simulink model "ASM_Traffic_MultiCore"  (R2026a)
settings: Solver=ode1  StartTime=SIM.tstart.v  StopTime=SIM.tend.v  FixedStep=SIM.StepSize.v
PostLoadFcn:
  | if any(exist('dsrtsu_mdlpostloadfcn', 'file') ~= 0), dsrtsu_mdlpostloadfcn('Execute', bdroot); end
  | try, asm_mdl_postloadfcn(bdroot, 'UpdateModel', 3600); catch, disp(lasterr); end,
InitFcn:
  | , if any(exist('rtifpga_mdlclblib', 'file') ~= 0), rtifpga_mdlclblib('Init', bdroot); end,
  | , if any(exist('dsmpb_private', 'file') ~= 0), dsmpb_private('dsmpb_mdlclblib', 'Init', bdroot); end,
model workspace (MAT data in the model file):
  asmReferencePath = [0 0.01 0.02 0.03 0.04 0.05 0.06 0.07 0.08 0.09 0.1 0.11 ... (350007 elements, 50001x7)]
  roadBounds : Simulink.Parameter (value not decoded)
  safetyAxes : Simulink.Parameter (value not decoded)
undefined symbols (not defined in the file): _to_, a0b2, ASM_BrakeHydraulics_DemoSystems, ASM_VehicleDynamics_DemoSystems, b98103fe8ad365046cd0, BrakeCircuit, controllerConfig, CPT, Crankshaft, DiscIntNeverNeededParam, dsmsi, FinalDriveAssembly, MDL, ModeSignals, mu, Pos_BrakePedal_Maneuver, rad, RefSignals, roadFamilyData, roadFamilyId, s_to_rpm, SIM, SoftECU, Suspension, Tire, Transmission
libraries: ASM_Traffic_lib x135, simulink x98, ASM_Utils_lib x77, ASM_VehicleDynamics_lib x70, ASM_Environment_lib x22, dsmpblib x20, dsmsilib x15, MDLD_Utils_lib x10, ASM_BrakeHydraulics_lib x3, sl_discontinuities x2
(part 2 of 65)

== system ASM_Traffic_MultiCore/ASMTools ==
  note: ---- Code Generation ----
  note: ------ Multi-Instance ------
  note: ----- Scope Handling ------
  note: ----- Signal Handling ------
  note: ------------------- Project & Experiment Handling -------------------
  note: -------------------- ModelDesk Parameter Group --------------------
  note: ------------------------------- Tire Handling -------------------------------
  ASMSignalInterface_Manager : MDLD_Utils_lib/ModelDeskPlotInterface/ASMSignalInterface_Manager
  ASM_Model_Port_Manager : ASM_Utils_lib/Miscellaneous/ASM_MODEL_PORT_MANAGER
  GenerateVEOS : ASM_Utils_lib/CodeGeneration/GenerateVEOS
  ModelDeskParaGroupOverview : ASM_Utils_lib/ModelDeskInterface/ModelDeskParaGroupOverview
  MultiInstanceOverview : ASM_Utils_lib/ModelDeskInterface/MultiInstanceOverview
  OpenExperimentModelDesk : ASM_Utils_lib/OpenExperiment/OpenExperiment  ExpDir=..\Parameterization\MOD_Traffic\Experiment_001\Experiment_001.CDE  dSProduct=ModelDesk
  ReplaceTire : ASM_Utils_lib/BlockReplacement/ReplaceVariants  editSearchPath=bdroot  popupLibBlk=<select here>  popupTargetDemo=<select here>  Demosystem=VehicleDynamics_Tire  variantLib=ASM_VehicleDynamics_DemoSystems/Tire
  ScopeHandlingGui : ASM_Utils_lib/ReplaceScopes/ScopeHandlingGui

== system ASM_Traffic_MultiCore/AnimationInterface ==
  note: Animation Interface
  In : Inport
  ANIMATION_INTERFACE : Subsystem
  Bus Selector : BusSelector  OutputSignals=Environment.Animation.Sw_AnimationInterface[0Disabled|1Enabled],Environment.Animation.ManeuverState[]
  DriverAssistance_Animation : BusSelector  OutputSignals=DomainControl.DriverAssistance.Animation  OutputAsBus=on
  Drivetrain_Animation : BusSelector  OutputSignals=Drivetrain.Animation  OutputAsBus=on
  Environment_Animation : BusSelector  OutputSignals=Environment.Animation  OutputAsBus=on
  FcnCall : Subsystem
  Fellow_Doors : Subsystem
  Fellow_Lights : Subsystem
  OpenAnimationInterfaceModel : Subsystem
      settings: OpenFcn=|
      | InterfaceModel = 'ASM_AnimationInterface';
      | 
      | try
      |     open_system(InterfaceModel);                         catch
      |     errordlg(['ERROR opening Animation interface: ',InterfaceModel,'.slx']);
      | end
      mask Display: disp('Open ASM_AnimationInterface')
  Rate Transition{,1..3} (4 alike) : RateTransition  Integrity=off  OutPortSampleTimeOpt=Inherit
  VehicleDynamics_Animation : BusSelector  OutputSignals=VehicleDynamics.Animation  OutputAsBus=on
  Vehicle_Doors : Subsystem
  Vehicle_Lights : Subsystem
  wires:
  Bus Selector/1 -> FcnCall/Enable  "<Sw_AnimationInterface[0Disabled|1Enabled]>"
  Fellow_Doors/1(Fellow_Doors) -> ANIMATION_INTERFACE/8(Fellow_Doors)
  Vehicle_Doors/1(ASM_Vehicle_Doors) -> ANIMATION_INTERFACE/7(ASM_Vehicle_Doors)
  Rate Transition2/1 -> ANIMATION_INTERFACE/4(Environment_Animation), Vehicle_Lights/2(Environment_Animation), Fellow_Doors/1(Environment_Animation), Vehicle_Doors/1(Environment_Animation), Fellow_Lights/1(Environment_Animation)
  Vehicle_Lights/1(ASM_Vehicle_Lights) -> ANIMATION_INTERFACE/5(ASM_Vehicle_Lights)
  Fellow_Lights/1(Fellow_Light) -> ANIMATION_INTERFACE/6(Fellow_Lights)
  Rate Transition3/1 -> ANIMATION_INTERFACE/3(VehicleDynamics_Animation), Vehicle_Lights/1(VehicleDynamics_Animation)
  FcnCall/1(FcnCallEvent[]) -> ANIMATION_INTERFACE/Trigger
  Bus Selector/2 -> FcnCall/1(ManeuverState[])  "<ManeuverState[]>"
  Drivetrain_Animation/1 -> Rate Transition1/1
  Rate Transition1/1 -> ANIMATION_INTERFACE/2(Drivetrain_Animation)
  Rate Transition/1 -> ANIMATION_INTERFACE/1(DriverAssistance_Animation)
  Environment_Animation/1 -> Rate Transition2/1
  DriverAssistance_Animation/1 -> Rate Transition/1
  VehicleDynamics_Animation/1 -> Rate Transition3/1
  In/1 -> VehicleDynamics_Animation/1, Environment_Animation/1, Drivetrain_Animation/1, DriverAssistance_Animation/1, Bus Selector/1

== system ASM_Traffic_MultiCore/DomainControl ==
  In : Inport
  Bus Creator : BusCreator  Inputs=3
  DriverAssistance : Subsystem
  StartSystem : Subsystem
  TorqueManager : Subsystem
  Out : Outport  VectorParamsAs1DForOutWhenUnconnected=off
  wires:
  Bus Creator/1 -> Out/1  "DomainControl"
  In/1 -> StartSystem/1(In), DriverAssistance/1(In), TorqueManager/1(In)
  DriverAssistance/1(Out) -> Bus Creator/3
  StartSystem/1(Out) -> Bus Creator/1
  TorqueManager/1(Out) -> Bus Creator/2

== system ASM_Traffic_MultiCore/Driver ==
  note: Driver
  In : Inport
  steering_wheel[deg] : Inport  Port=2
  Interface_In : Subsystem
  Interface_Out : Subsystem
  Plant : Subsystem
  SignalInterface : Subsystem
  Out : Outport  VectorParamsAs1DForOutWhenUnconnected=off
  wires:
  In/1 -> Interface_In/1(In)
  Interface_In/1(Out) -> SignalInterface/1(In), Plant/1(Interface_In)
  Plant/1(Plant) -> Interface_Out/1(In)
  Interface_Out/1(Out) -> Out/1
  steering_wheel[deg]/1 -> Plant/2(steering_wheel[deg])

== system ASM_Traffic_MultiCore/Drivetrain ==
  note: Drivetrain
  In : Inport
  drive_trq[Nm] : Inport  Port=2
  Bus Creator1 : BusCreator  Inputs=2
  Control : Subsystem
  Interface_In : Subsystem
  Interface_Out : Subsystem
  Plant : Subsystem
  SignalInterface : Subsystem
  Out : Outport  VectorParamsAs1DForOutWhenUnconnected=off
  wires:
  Control/1(Control) -> Plant/2(Control), Bus Creator1/2
  Plant/1(Plant) -> Control/2(Plant), Bus Creator1/1
  Bus Creator1/1 -> Interface_Out/1(In)
  In/1 -> Interface_In/1(In)
  Interface_Out/1(Out) -> Out/1
  Interface_In/1(Out) -> SignalInterface/1(In), Control/1(Interface_In), Plant/1(Interface_In)
  drive_trq[Nm]/1 -> Plant/3(drive_trq[Nm])

== system ASM_Traffic_MultiCore/ElectricalSystem ==
  note: Electrical System Basic
  In : Inport
  Bus Creator2 : BusCreator  Inputs=2
  Control : Subsystem
  Interface_In : Subsystem
  Interface_Out : Subsystem
  Plant : Subsystem
  SignalInterface : Subsystem
  Out : Outport  VectorParamsAs1DForOutWhenUnconnected=off
  wires:
  Bus Creator2/1 -> Interface_Out/1(In)
  Control/1(Control) -> Plant/2(Control), Bus Creator2/2
  In/1 -> Interface_In/1(In)
  Plant/1(Plant) -> Control/2(Plant), Bus Creator2/1
  Interface_Out/1(Out) -> Out/1
  Interface_In/1(Out) -> SignalInterface/1(In), Control/1(Interface_In), Plant/1(Interface_In)

== system ASM_Traffic_MultiCore/Engine ==
  note: Engine Basic
  In : Inport
  Bus Creator1 : BusCreator  Inputs=2
  Control : Subsystem
  Interface_In : Subsystem
  Interface_Out : Subsystem
  Plant : Subsystem
  SignalInterface : Subsystem
  Out : Outport  VectorParamsAs1DForOutWhenUnconnected=off
  wires:
  In/1 -> Interface_In/1(In)
  Interface_Out/1(Out) -> Out/1
  Control/1(Control) -> Plant/2(Control), Bus Creator1/2
  Interface_In/1(Out) -> SignalInterface/1(In), Control/1(Interface_In), Plant/1(Interface_In)
  Plant/1(Plant) -> Bus Creator1/1, Control/2(Plant)
  Bus Creator1/1 -> Interface_Out/1(In)

== system ASM_Traffic_MultiCore/Environment ==
  note: Environment Traffic
  In : Inport
  Bus Creator1 : BusCreator  Inputs=6
  GroundTruth : Subsystem
  Interface_In : Subsystem
  Interface_Out : Subsystem
  Maneuver : Subsystem
  ModelDesk_MC_ID_Environment : ASM_Utils_lib/ModelDeskInterface/ModelDesk_MC  Tag=ASM_MAINCOMPONENT  Editable=off  MainComponent=Environment
  Road : Subsystem
  Sensors : Subsystem
  SignalInterface : Subsystem
  Traffic : Subsystem
  Out : Outport  VectorParamsAs1DForOutWhenUnconnected=off
  wires:
  In/1 -> Interface_In/1(In)
  GroundTruth/1(Out) -> Bus Creator1/6
  Sensors/1(Out) -> Bus Creator1/5
  Interface_In/1(Out) -> Bus Creator1/1
  Bus Creator1/1 -> SignalInterface/1(In), Sensors/1(In), Traffic/1(In), Road/1(In), Maneuver/1(In), GroundTruth/1(In), Interface_Out/1(In)
  Traffic/1(Out) -> Bus Creator1/4
  Road/1(Out) -> Bus Creator1/3
  Maneuver/1(Out) -> Bus Creator1/2
  Interface_Out/1(Out) -> Out/1

== system ASM_Traffic_MultiCore/Help ==

== system ASM_Traffic_MultiCore/VehicleDynamics ==
  note: Vehicle Dynamics
  In : Inport
  Ext_BrakeTrq[Nm] : Inport  Port=2
  deltaF_cmd_deg : Inport  Port=3
  Bus Creator1 : BusCreator  Inputs=2
  Control : Subsystem
  Interface_In : Subsystem
  Interface_Out : Subsystem
  Plant : Subsystem
  SignalInterface : Subsystem
  Out : Outport  VectorParamsAs1DForOutWhenUnconnected=off
  F_y[N] : Outport  Port=2
  F_z[N] : Outport  Port=3
  wires:
  Interface_Out/1(Out) -> Out/1
  In/1 -> Interface_In/1(In)
  Plant/1(Plant) -> Bus Creator1/1, Control/2(Plant)
  Control/1(Control) -> Plant/4(Control), Bus Creator1/2
  Interface_In/1(Out) -> SignalInterface/1(In), Control/1(Interface_In), Plant/3(Interface_In)
  Bus Creator1/1 -> Interface_Out/1(In)
  Ext_BrakeTrq[Nm]/1 -> Plant/2(Ext_BrakeTrq[Nm])
  Plant/2(F_y[N]) -> F_y[N]/1
  Plant/3(F_z[N]) -> F_z[N]/1
  deltaF_cmd_deg/1 -> Plant/1(deltaF_cmd_deg)

== system ASM_Traffic_MultiCore/controller_subsys ==
  In Bus Element : Inport  PortName=measurements  Element=x
  BusElementIn2 : Inport  PortName=measurements  Element=vx
  BusElementIn : Inport  PortName=measurements  Element=s
  horizon_prep_in : Inport  Port=2
  fellow : Inport  Port=3
  In Bus Element2 : Inport  Port=4  PortName=execution
  Reshape : Reshape  OutputDimensionality=Customize  OutputDimensions=[205,1]
  Terminator : Terminator
  Unit Delay : UnitDelay  SampleTime=0.05
  Unit Delay1 : UnitDelay  SampleTime=0.05
  acados_solver : Subsystem
  assemble_problem : MATLAB Function  TreatAsAtomicUnit=on
  horizon_prep : MATLAB Function  TreatAsAtomicUnit=on
  input_prep : Subsystem
  output_routing : Subsystem
  warm_start : Subsystem
  Out Bus Element : Outport  PortName=command
  Out Bus Element1 : Outport  Port=2  PortName=telemetry
  wires:
  acados_solver/1(solver_outputs) -> output_routing/1(solver_outputs)
  In Bus Element/1 -> assemble_problem/1(x)
  assemble_problem/1(solverInputs) -> input_prep/1(InBus)
  output_routing/2(predictions) -> warm_start/1(predictions)
  warm_start/1(x_pred) -> Unit Delay/1
  warm_start/2(u_pred) -> Unit Delay1/1
  input_prep/1(solverInputs) -> acados_solver/1(solverInputs)  "replay"
  horizon_prep/1(P) -> assemble_problem/2(P)
  BusElementIn2/1 -> horizon_prep/2(vx)
  BusElementIn/1 -> horizon_prep/1(s)
  output_routing/1(command) -> Out Bus Element/1
  output_routing/3(telemetry) -> Out Bus Element1/1
  In Bus Element2/1 -> input_prep/2(InBus1)
  Unit Delay/1 -> assemble_problem/3(Xguess), Reshape/1
  Unit Delay1/1 -> assemble_problem/4(Uguess)
  Reshape/1 -> horizon_prep/4(Xguess)
  horizon_prep_in/1 -> Terminator/1
  fellow/1 -> horizon_prep/3(fellow)

== system ASM_Traffic_MultiCore/exec_setting ==
  Constant : Constant  Value=false  OutDataTypeStr=boolean
  Constant1 : Constant  Value=true  OutDataTypeStr=boolean
  Constant2 : Constant  Value=200
  Out Bus Element : Outport  PortName=execution  Element=reset
  BusElementOut : Outport  PortName=execution  Element=enable
  BusElementOut1 : Outport  PortName=execution  Element=cap
  wires:
  Constant/1 -> Out Bus Element/1
  Constant1/1 -> BusElementOut/1
  Constant2/1 -> BusElementOut1/1

== system ASM_Traffic_MultiCore/state_conversion ==
  In4 : Inport
  F_y[N] : Inport  Port=2
  F_z[N] : Inport  Port=3
  ASM_adapter : MATLAB Function  TreatAsAtomicUnit=on
  Angle_fl_fr_wheel_vector : Concatenate
  Bus Selector : BusSelector  OutputSignals=x,vx,s
  Constant : Constant  Value=0
  Gain : Gain  Gain=1/3.6
  Gain1 : Gain  Gain=1/3.6
  Horizon_prep_in_vector : Concatenate  NumInputs=4
  Kinematic_sI_vector : Concatenate  NumInputs=4
  Reference_SI_vector : Concatenate  NumInputs=7
  Terminator{,2,5..6} (4 alike) : Terminator
  deg2rad : Gain  Gain=pi/180
  deg2rad1 : Gain  Gain=pi/180
  deg2rad2 : Gain  Gain=pi/180
  fellow_vector : Concatenate  NumInputs=4
  measured_pos : Concatenate
  required_measurement : BusSelector  OutputSignals=VehicleDynamics.Plant.v_x_Vehicle_CoG[km|h],VehicleDynamics.Plant.v_y_Vehicle_CoG[km|h],VehicleDynamics.Plant.Angle_Yaw_Vehicle_CoorSys_E[deg],VehicleDynamics.Plant.YawRate_Vehicle_CoG[deg|s],VehicleDynamics.Plant.Pos_x_Vehicle_CoorSys_E[m],VehicleDynamics.Plant.Pos_y_Vehicle_CoorSys_E[m],VehicleDynamics.Plant.Angle_SteeringWheel[deg],Environment.Plant.Pos_x_Ref_Vehicle_Road[m],Environment.Plant.Pos_y_Ref_Vehicle_Road[m],Environment.Plant.Curv_Vehicle_Road[1|m],Environment.Plant.s_Total_Vehicle_Road[m],Environment.Plant.s_Vehicle_Road[m],Environment.Plant.Angle_Yaw_Veh_Road[deg],Environment.Plant.v_Vehicle_Ref_Maneuver[m|s],Environment.Plant.v_Vehicle_Preview_Ref_Maneuver[m|s],Environment.Plant.Curv_Preview_Road[1|m],Driver.Plant.s_Preview[m],Environment.Plant.Pos_y_Preview_Road[m],Environment.Plant.Pos_x_Preview_Road[m],Environment.Plant.d_Total_Fellows[m],Environment.Plant.s_Fellows_Ref[m],Environment.Animation.Flag_FellowUsed[0|1],Environment.Animation.v_Fellows[km|h],Environment.Plant.Fric_Coeff_CP[:][],VehicleDynamics.Plant.Trq_Max_Brake[Nm],VehicleDynamics.Animation.F_FL_Tire_CoorSys_V[x;y;z][N],VehicleDynamics.Animation.F_FR_Tire_CoorSys_V[x;y;z][N],VehicleDynamics.Animation.F_RL_Tire_CoorSys_V[x;y;z][N],VehicleDynamics.Animation.F_RR_Tire_CoorSys_V[x;y;z][N],VehicleDynamics.Animation.Angle_FL_Wheel[Toe;Camber][deg],VehicleDynamics.Animation.Angle_FR_Wheel[Toe;Camber][deg]
  tire_feature_vector : Concatenate  NumInputs=6
  BusElementOut : Outport  PortName=measurement  Element=x
  BusElementOut1 : Outport  PortName=measurement  Element=vx
  Out Bus Element : Outport  PortName=measurement  Element=s
  horizon_prep_in : Outport  Port=2
  fellow : Outport  Port=3
  FyWheel[N] : Outport  Port=4
  FzWheel : Outport  Port=5
  tire_feature : Outport  Port=6
  Angle_FL_FR_Wheel[Toe;Camber][deg] : Outport  Port=7
  wires:
  Gain1/1 -> Kinematic_sI_vector/2
  required_measurement/5 -> measured_pos/1  "<Pos_x_Vehicle_CoorSys_E[m]>"
  required_measurement/9 -> Reference_SI_vector/2  "<Pos_y_Ref_Vehicle_Road[m]>"
  required_measurement/7 -> Terminator/1  "<Angle_SteeringWheel[deg]>"
  deg2rad1/1 -> Kinematic_sI_vector/4
  required_measurement/3 -> deg2rad/1  "<Angle_Yaw_Vehicle_CoorSys_E[deg]>"
  measured_pos/1 -> ASM_adapter/2(vehicleXY)
  Gain/1 -> Kinematic_sI_vector/1
  Kinematic_sI_vector/1 -> ASM_adapter/1(kinematicsSI)
  required_measurement/4 -> deg2rad1/1  "<YawRate_Vehicle_CoG[deg|s]>"
  required_measurement/6 -> measured_pos/2  "<Pos_y_Vehicle_CoorSys_E[m]>"
  required_measurement/1 -> Gain/1  "<v_x_Vehicle_CoG[km|h]>"
  deg2rad/1 -> Kinematic_sI_vector/3
  ASM_adapter/1(measurement) -> Bus Selector/1
  required_measurement/2 -> Gain1/1  "<v_y_Vehicle_CoG[km|h]>"
  required_measurement/8 -> Reference_SI_vector/1  "<Pos_x_Ref_Vehicle_Road[m]>"
  In4/1 -> required_measurement/1
  Reference_SI_vector/1 -> ASM_adapter/3(referenceSI)
  Bus Selector/1 -> BusElementOut/1  "<x>"
  Bus Selector/2 -> BusElementOut1/1  "<vx>"
  Bus Selector/3 -> Out Bus Element/1  "<s>"
  required_measurement/12 -> Terminator2/1  "<s_Vehicle_Road[m]>"
  required_measurement/11 -> Reference_SI_vector/3  "<s_Total_Vehicle_Road[m]>"
  required_measurement/10 -> Reference_SI_vector/5  "<Curv_Vehicle_Road[1|m]>"
  required_measurement/19 -> Terminator6/1  "<Pos_x_Preview_Road[m]>"
  required_measurement/18 -> Terminator5/1  "<Pos_y_Preview_Road[m]>"
  required_measurement/16 -> Horizon_prep_in_vector/3  "<Curv_Preview_Road[1|m]>"
  required_measurement/13 -> deg2rad2/1  "<Angle_Yaw_Veh_Road[deg]>"
  required_measurement/14 -> Reference_SI_vector/7, Horizon_prep_in_vector/1  "<v_Vehicle_Ref_Maneuver[m|s]>"
  required_measurement/15 -> Horizon_prep_in_vector/2  "<v_Vehicle_Preview_Ref_Maneuver[m|s]>"
  Constant/1 -> Reference_SI_vector/6
  deg2rad2/1 -> Reference_SI_vector/4
  required_measurement/17 -> Horizon_prep_in_vector/4  "<s_Preview[m]>"
  Horizon_prep_in_vector/1 -> horizon_prep_in/1
  required_measurement/20 -> fellow_vector/1  "<d_Total_Fellows[m]>"
  required_measurement/21 -> fellow_vector/2  "<s_Fellows_Ref[m]>"
  required_measurement/22 -> fellow_vector/3  "<Flag_FellowUsed[0|1]>"
  required_measurement/23 -> fellow_vector/4  "<v_Fellows[km|h]>"
  fellow_vector/1 -> fellow/1
  required_measurement/24 -> tire_feature_vector/1  "<Fric_Coeff_CP[:][]>"
  required_measurement/25 -> tire_feature_vector/2  "<Trq_Max_Brake[Nm]>"
  required_measurement/26 -> tire_feature_vector/3  "<F_FL_Tire_CoorSys_V[x;y;z][N]>"
  required_measurement/27 -> tire_feature_vector/4  "<F_FR_Tire_CoorSys_V[x;y;z][N]>"
  required_measurement/28 -> tire_feature_vector/5  "<F_RL_Tire_CoorSys_V[x;y;z][N]>"
  required_measurement/29 -> tire_feature_vector/6  "<F_RR_Tire_CoorSys_V[x;y;z][N]>"
  tire_feature_vector/1 -> tire_feature/1
  F_z[N]/1 -> FzWheel/1
  F_y[N]/1 -> FyWheel[N]/1
  required_measurement/30 -> Angle_fl_fr_wheel_vector/1  "<Angle_FL_Wheel[Toe;Camber][deg]>"
  required_measurement/31 -> Angle_fl_fr_wheel_vector/2  "<Angle_FR_Wheel[Toe;Camber][deg]>"
  Angle_fl_fr_wheel_vector/1 -> Angle_FL_FR_Wheel[Toe;Camber][deg]/1

== system ASM_Traffic_MultiCore/telemetry_unwrapped ==
  In1 : Inport
  Bus Selector : BusSelector  OutputSignals=slack_values,solver_status,cost_value,kkt_residuals,cpu_time,cpu_time_qp,cpu_time_lin,sqp_iter,qp_iteration_history,residual_history,history_length,lam_stage0
  Terminator{,1..11} (12 alike) : Terminator
  history_length : SignalConversion  OverrideOpt=off
  kkt_residuals : SignalConversion  OverrideOpt=off
  lam_stage0 : SignalConversion  OverrideOpt=off
  linearization_time_s : SignalConversion  OverrideOpt=off
  qp_iteration_history : SignalConversion  OverrideOpt=off
  qp_time_s : SignalConversion  OverrideOpt=off
  residual_history : SignalConversion  OverrideOpt=off
  slack_values : SignalConversion  OverrideOpt=off
  solver_cost : SignalConversion  OverrideOpt=off
  solver_status : SignalConversion  OverrideOpt=off
  solver_time_s : SignalConversion  OverrideOpt=off
  sqp_iterations : SignalConversion  OverrideOpt=off
  wires:
  Bus Selector/1 -> slack_values/1  "<slack_values>"
  Bus Selector/9 -> qp_iteration_history/1  "<qp_iteration_history>"
  Bus Selector/12 -> lam_stage0/1  "<lam_stage0>"
  Bus Selector/10 -> residual_history/1  "<residual_history>"
  Bus Selector/11 -> history_length/1  "<history_length>"
  In1/1 -> Bus Selector/1
  Bus Selector/2 -> solver_status/1  "<solver_status>"
  solver_status/1 -> Terminator1/1  "solver_status"
  Bus Selector/3 -> solver_cost/1  "<cost_value>"
  solver_cost/1 -> Terminator2/1  "solver_cost"
  Bus Selector/4 -> kkt_residuals/1  "<kkt_residuals>"
  kkt_residuals/1 -> Terminator3/1  "kkt_residuals"
  Bus Selector/5 -> solver_time_s/1  "<cpu_time>"
  solver_time_s/1 -> Terminator4/1  "solver_time_s"
  Bus Selector/6 -> qp_time_s/1  "<cpu_time_qp>"
  qp_time_s/1 -> Terminator5/1  "qp_time_s"
  Bus Selector/7 -> linearization_time_s/1  "<cpu_time_lin>"
  linearization_time_s/1 -> Terminator6/1  "linearization_time_s"
  Bus Selector/8 -> sqp_iterations/1  "<sqp_iter>"
  sqp_iterations/1 -> Terminator7/1  "sqp_iterations"
  slack_values/1 -> Terminator/1  "slack_values"
  qp_iteration_history/1 -> Terminator8/1
  residual_history/1 -> Terminator9/1
  lam_stage0/1 -> Terminator11/1
  history_length/1 -> Terminator10/1

== system ASM_Traffic_MultiCore/AnimationInterface/ANIMATION_INTERFACE ==
  DriverAssistance_Animation : Inport
  Drivetrain_Animation : Inport  Port=2
  VehicleDynamics_Animation : Inport  Port=3
  Environment_Animation : Inport  Port=4
  ASM_Vehicle_Lights : Inport  Port=5
  Fellow_Lights : Inport  Port=6
  ASM_Vehicle_Doors : Inport  Port=7
  Fellow_Doors : Inport  Port=8
  function : TriggerPort  TriggerType=function-call  VariantControl=Variant
  ACC_Instruments : Subsystem  Tag=Animation_ACC_Instruments  Priority=10001  Commented=on
  ASM_Vehicle : Subsystem  Tag=Animation_ASM_Vehicle  Priority=10001
  ASM_Vehicle_Instruments : Subsystem  Tag=Animation_ASM_Vehicle_Instruments  Priority=10001
  ASM_Vehicle_Occupants : Subsystem  Tag=Animation_ASM_Vehicle_Occupants  Priority=10001
  Activate_Animation : Subsystem  mask{ASMVehicle=Uncomment, ASMVehicleInstruments=Uncomment, ASMSensors=Uncomment, BoundigBoxes=Uncomment}
      mask prompts: ASMVehicle "ASM Vehicle"; ASMVehicleInstruments "ASM Vehicle Instruments"; ASMSensors "ASM Sensors"; BoundigBoxes "Bounding Boxes"
      settings: OpenFcn=|
      | subsysTag = 'Animation_Bounding_Boxes';
      | subsys = find_system(get_param(gcb,'Parent'),'SearchDepth','1','IncludeCommented','on','Tag',subsysTag);
      | if ~isempty(subsys)
      |     subsysState = get_param(subsys,'commented');
      |     if strcmp(subsysState,'off')
      |         set_param(subsys{1},'commented','on')
      |     end
      |     if strcmp(subsysState,'on')
      |         set_param(subsys{1},'commented','off')
      |     end
      | else
      |     disp(['Subsystem tagged with ''', subsysTag, ''' could not be found. The button is without action.'])
      | end
      mask TypeOptions ASMVehicle: Comment out | Uncomment
      mask Callback ASMVehicle: asm_vehicle_comment(gcb)
      mask TypeOptions ASMVehicleInstruments: Comment out | Uncomment
      mask TypeOptions ASMSensors: Comment out | Uncomment
      mask Callback ASMSensors:
      | subsys = find_system(get_param(gcb,'Parent'),'SearchDepth','1','IncludeCommented','on','Tag','ASM_Sensors');
      | if ~isempty(subsys)
      |     button_state = get_param(gcb,'ASMSensors');
      |     subsys_state = get_param(subsys,'commented');
      |     if strcmp(button_state,'Comment out') && strcmp(subsys_state,'off')
      |         set_param(subsys{1},'commented','on')
      |     end
      |     if strcmp(button_state,'Uncomment') && strcmp(subsys_state,'on')
      |         set_param(subsys{1},'commented','off')
      |     end
      | end
      mask TypeOptions BoundigBoxes: Comment out | Uncomment
      mask Display: disp('double click to\n activate/deactivate')
  Activate_Animation1 : Subsystem  mask{ASMVehicle=Uncomment, ASMVehicleInstruments=Uncomment, ASMSensors=Uncomment, BoundigBoxes=Uncomment}
      mask prompts: ASMVehicle "ASM Vehicle"; ASMVehicleInstruments "ASM Vehicle Instruments"; ASMSensors "ASM Sensors"; BoundigBoxes "Bounding Boxes"
      settings: OpenFcn=|
      | subsysTag = 'Animation_Fellows';
      | subsys = find_system(get_param(gcb,'Parent'),'SearchDepth','1','IncludeCommented','on','Tag',subsysTag);
      | if ~isempty(subsys)
      |     subsysState = get_param(subsys,'commented');
      |     if strcmp(subsysState,'off')
      |         set_param(subsys{1},'commented','on')
      |     end
      |     if strcmp(subsysState,'on')
      |         set_param(subsys{1},'commented','off')
      |     end
      | else
      |     disp(['Subsystem tagged with ''', subsysTag, ''' could not be found. The button is without action.'])
      | end
      mask TypeOptions ASMVehicle: Comment out | Uncomment
      mask Callback ASMVehicle: asm_vehicle_comment(gcb)
      mask TypeOptions ASMVehicleInstruments: Comment out | Uncomment
      mask TypeOptions ASMSensors: Comment out | Uncomment
      mask Callback ASMSensors:
      | subsys = find_system(get_param(gcb,'Parent'),'SearchDepth','1','IncludeCommented','on','Tag','ASM_Sensors');
      | if ~isempty(subsys)
      |     button_state = get_param(gcb,'ASMSensors');
      |     subsys_state = get_param(subsys,'commented');
      |     if strcmp(button_state,'Comment out') && strcmp(subsys_state,'off')
      |         set_param(subsys{1},'commented','on')
      |     end
      |     if strcmp(button_state,'Uncomment') && strcmp(subsys_state,'on')
      |         set_param(subsys{1},'commented','off')
      |     end
      | end
      mask TypeOptions BoundigBoxes: Comment out | Uncomment
      mask Display: disp('double click to\n activate/deactivate')
  Activate_Animation2 : Subsystem  mask{ASMVehicle=Uncomment, ASMVehicleInstruments=Uncomment, ASMSensors=Uncomment, BoundigBoxes=Uncomment}
      mask prompts: ASMVehicle "ASM Vehicle"; ASMVehicleInstruments "ASM Vehicle Instruments"; ASMSensors "ASM Sensors"; BoundigBoxes "Bounding Boxes"
      settings: OpenFcn=|
      | subsysTag = 'Animation_Data_Streams_Instruments';
      | subsys = find_system(get_param(gcb,'Parent'),'SearchDepth','1','IncludeCommented','on','Tag',subsysTag);
      | if ~isempty(subsys)
      |     subsysState = get_param(subsys,'commented');
      |     if strcmp(subsysState,'off')
      |         set_param(subsys{1},'commented','on')
      |     end
      |     if strcmp(subsysState,'on')
      |         set_param(subsys{1},'commented','off')
      |     end
      | else
      |     disp(['Subsystem tagged with ''', subsysTag, ''' could not be found. The button is without action.'])
      | end
      mask TypeOptions ASMVehicle: Comment out | Uncomment
      mask Callback ASMVehicle: asm_vehicle_comment(gcb)
      mask TypeOptions ASMVehicleInstruments: Comment out | Uncomment
      mask TypeOptions ASMSensors: Comment out | Uncomment
      mask Callback ASMSensors:
      | subsys = find_system(get_param(gcb,'Parent'),'SearchDepth','1','IncludeCommented','on','Tag','ASM_Sensors');
      | if ~isempty(subsys)
      |     button_state = get_param(gcb,'ASMSensors');
      |     subsys_state = get_param(subsys,'commented');
      |     if strcmp(button_state,'Comment out') && strcmp(subsys_state,'off')
      |         set_param(subsys{1},'commented','on')
      |     end
      |     if strcmp(button_state,'Uncomment') && strcmp(subsys_state,'on')
      |         set_param(subsys{1},'commented','off')
      |     end
      | end
      mask TypeOptions BoundigBoxes: Comment out | Uncomment
      mask Display: disp('double click to\n activate/deactivate')
  Activate_Animation3 : Subsystem  mask{ASMVehicle=Uncomment, ASMVehicleInstruments=Uncomment, ASMSensors=Uncomment, BoundigBoxes=Uncomment}
      mask prompts: ASMVehicle "ASM Vehicle"; ASMVehicleInstruments "ASM Vehicle Instruments"; ASMSensors "ASM Sensors"; BoundigBoxes "Bounding Boxes"
      settings: OpenFcn=|
      | subsysTag = 'Animation_Lane_Sensor';
      | subsys = find_system(get_param(gcb,'Parent'),'SearchDepth','1','IncludeCommented','on','Tag',subsysTag);
      | if ~isempty(subsys)
      |     subsysState = get_param(subsys,'commented');
      |     if strcmp(subsysState,'off')
      |         set_param(subsys{1},'commented','on')
      |     end
      |     if strcmp(subsysState,'on')
      |         set_param(subsys{1},'commented','off')
      |     end
      | else
      |     disp(['Subsystem tagged with ''', subsysTag, ''' could not be found. The button is without action.'])
      | end
      mask TypeOptions ASMVehicle: Comment out | Uncomment
      mask Callback ASMVehicle: asm_vehicle_comment(gcb)
      mask TypeOptions ASMVehicleInstruments: Comment out | Uncomment
      mask TypeOptions ASMSensors: Comment out | Uncomment
      mask Callback ASMSensors:
      | subsys = find_system(get_param(gcb,'Parent'),'SearchDepth','1','IncludeCommented','on','Tag','ASM_Sensors');
      | if ~isempty(subsys)
      |     button_state = get_param(gcb,'ASMSensors');
      |     subsys_state = get_param(subsys,'commented');
      |     if strcmp(button_state,'Comment out') && strcmp(subsys_state,'off')
      |         set_param(subsys{1},'commented','on')
      |     end
      |     if strcmp(button_state,'Uncomment') && strcmp(subsys_state,'on')
      |         set_param(subsys{1},'commented','off')
      |     end
      | end
      mask TypeOptions BoundigBoxes: Comment out | Uncomment
      mask Display: disp('double click to\n activate/deactivate')
  Activate_Animation4 : Subsystem  mask{ASMVehicle=Uncomment, ASMVehicleInstruments=Uncomment, ASMSensors=Uncomment, BoundigBoxes=Uncomment}
      mask prompts: ASMVehicle "ASM Vehicle"; ASMVehicleInstruments "ASM Vehicle Instruments"; ASMSensors "ASM Sensors"; BoundigBoxes "Bounding Boxes"
      settings: OpenFcn=|
      | subsysTag = 'Animation_Lane_Sensor_Dynamic_Instruments';
      | subsys = find_system(get_param(gcb,'Parent'),'SearchDepth','1','IncludeCommented','on','Tag',subsysTag);
      | if ~isempty(subsys)
      |     subsysState = get_param(subsys,'commented');
      |     if strcmp(subsysState,'off')
      |         set_param(subsys{1},'commented','on')
      |     end
      |     if strcmp(subsysState,'on')
      |         set_param(subsys{1},'commented','off')
      |     end
      | else
      |     disp(['Subsystem tagged with ''', subsysTag, ''' could not be found. The button is without action.'])
      | end
      mask TypeOptions ASMVehicle: Comment out | Uncomment
      mask Callback ASMVehicle: asm_vehicle_comment(gcb)
      mask TypeOptions ASMVehicleInstruments: Comment out | Uncomment
      mask TypeOptions ASMSensors: Comment out | Uncomment
      mask Callback ASMSensors:
      | subsys = find_system(get_param(gcb,'Parent'),'SearchDepth','1','IncludeCommented','on','Tag','ASM_Sensors');
      | if ~isempty(subsys)
      |     button_state = get_param(gcb,'ASMSensors');
      |     subsys_state = get_param(subsys,'commented');
      |     if strcmp(button_state,'Comment out') && strcmp(subsys_state,'off')
      |         set_param(subsys{1},'commented','on')
      |     end
      |     if strcmp(button_state,'Uncomment') && strcmp(subsys_state,'on')
      |         set_param(subsys{1},'commented','off')
      |     end
      | end
      mask TypeOptions BoundigBoxes: Comment out | Uncomment
      mask Display: disp('double click to\n activate/deactivate')
  Activate_Animation5 : Subsystem  mask{ASMVehicle=Uncomment, ASMVehicleInstruments=Uncomment, ASMSensors=Uncomment, BoundigBoxes=Uncomment}
      mask prompts: ASMVehicle "ASM Vehicle"; ASMVehicleInstruments "ASM Vehicle Instruments"; ASMSensors "ASM Sensors"; BoundigBoxes "Bounding Boxes"
      settings: OpenFcn=|
      | subsysTag = 'Animation_ACC_Instruments';
      | subsys = find_system(get_param(gcb,'Parent'),'SearchDepth','1','IncludeCommented','on','Tag',subsysTag);
      | if ~isempty(subsys)
      |     subsysState = get_param(subsys,'commented');
      |     if strcmp(subsysState,'off')
      |         set_param(subsys{1},'commented','on')
      |     end
      |     if strcmp(subsysState,'on')
      |         set_param(subsys{1},'commented','off')
      |     end
      | else
      |     disp(['Subsystem tagged with ''', subsysTag, ''' could not be found. The button is without action.'])
      | end
      mask TypeOptions ASMVehicle: Comment out | Uncomment
      mask Callback ASMVehicle: asm_vehicle_comment(gcb)
      mask TypeOptions ASMVehicleInstruments: Comment out | Uncomment
      mask TypeOptions ASMSensors: Comment out | Uncomment
      mask Callback ASMSensors:
      | subsys = find_system(get_param(gcb,'Parent'),'SearchDepth','1','IncludeCommented','on','Tag','ASM_Sensors');
      | if ~isempty(subsys)
      |     button_state = get_param(gcb,'ASMSensors');
      |     subsys_state = get_param(subsys,'commented');
      |     if strcmp(button_state,'Comment out') && strcmp(subsys_state,'off')
      |         set_param(subsys{1},'commented','on')
      |     end
      |     if strcmp(button_state,'Uncomment') && strcmp(subsys_state,'on')
      |         set_param(subsys{1},'commented','off')
      |     end
      | end
      mask TypeOptions BoundigBoxes: Comment out | Uncomment
      mask Display: disp('double click to\n activate/deactivate')
  Activate_Animation6 : Subsystem  mask{ASMVehicle=Uncomment, ASMVehicleInstruments=Uncomment, ASMSensors=Uncomment, BoundigBoxes=Uncomment}
      mask prompts: ASMVehicle "ASM Vehicle"; ASMVehicleInstruments "ASM Vehicle Instruments"; ASMSensors "ASM Sensors"; BoundigBoxes "Bounding Boxes"
      settings: OpenFcn=|
      | subsysTag = 'Animation_Sensors';
      | subsys = find_system(get_param(gcb,'Parent'),'SearchDepth','1','IncludeCommented','on','Tag',subsysTag);
      | if ~isempty(subsys)
      |     subsysState = get_param(subsys,'commented');
      |     if strcmp(subsysState,'off')
      |         set_param(subsys{1},'commented','on')
      |     end
      |     if strcmp(subsysState,'on')
      |         set_param(subsys{1},'commented','off')
      |     end
      | else
      |     disp(['Subsystem tagged with ''', subsysTag, ''' could not be found. The button is without action.'])
      | end
      mask TypeOptions ASMVehicle: Comment out | Uncomment
      mask Callback ASMVehicle: asm_vehicle_comment(gcb)
      mask TypeOptions ASMVehicleInstruments: Comment out | Uncomment
      mask TypeOptions ASMSensors: Comment out | Uncomment
      mask Callback ASMSensors:
      | subsys = find_system(get_param(gcb,'Parent'),'SearchDepth','1','IncludeCommented','on','Tag','ASM_Sensors');
      | if ~isempty(subsys)
      |     button_state = get_param(gcb,'ASMSensors');
      |     subsys_state = get_param(subsys,'commented');
      |     if strcmp(button_state,'Comment out') && strcmp(subsys_state,'off')
      |         set_param(subsys{1},'commented','on')
      |     end
      |     if strcmp(button_state,'Uncomment') && strcmp(subsys_state,'on')
      |         set_param(subsys{1},'commented','off')
      |     end
      | end
      mask TypeOptions BoundigBoxes: Comment out | Uncomment
      mask Display: disp('double click to\n activate/deactivate')
  Bounding_Boxes : Subsystem  Tag=Animation_Bounding_Boxes  Priority=10001
  Connection_Settings : Subsystem  Tag=AnimationInterface_Connection_Settings  Priority=10009  mask(Connection_Settings){CommunicationMethod=Communication Service, Sw_Mode=0, ModelStepSize=SIM.StepSize.v, NumSamples=SIM.NumSamplesAnimation.v, MaxMessageSize=65507}
      mask prompts: CommunicationMethod "Communication method"; Sw_Mode "Simulation mode [0SIL|1HIL]"; ModelStepSize "Step size of the model [s]"; NumSamples "Time steps between two sent messages []"; MaxMessageSize "Maximum message size [bytes]"
      mask help: Specifies the communication method for transferring the collected simulation data to a consuming application.
      mask TypeOptions CommunicationMethod: Ethernet TCP | Communication Service
      mask Callback CommunicationMethod:
      | CommunicationMethod = Simulink.Mask.get(gcb).getParameter('CommunicationMethod'); % Ethernet TCP; Communication Service
      | 
      |     % Get Mask Dialogs & Controls
      |     EthernetTCPDescription      = Simulink.Mask.get(gcb).getDialogControl('EthernetTCPDescription');
      |     COMServiceDescription       = Simulink.Mask.get(gcb).getDialogControl('COMServiceDescription');
      |     AdvancedSettingsContainer   = Simulink.Mask.get(gcb).getDialogControl('AdvancedSettings');
      | 
      |     % Get Ethernet TCP Parameter
      |     Sw_Mode                     = Simulink.Mask.get(gcb).getParameter('Sw_Mode'); % SIL or HIL
      | 
      |     % Get Communication Service Parameter
      |     ModelStepSize               = Simulink.Mask.get(gcb).getParameter('ModelStepSize');
      |     NumSamples                  = Simulink.Mask.get(gcb).getParameter('NumSamples');
      |     MaxMessageSize              = Simulink.Mask.get(gcb).getParameter('MaxMessageSize');
      | 
      |     % Get blocks inside the masked subsystem
      |     SwCommunicationMethod           = [gcb,'/Sw_CommunicationMethod[0TCP|1ComService]'];     % Constant block for switching the Communication Method
      |     SubSysEthernetTCP               = [gcb,'/Ethernet_TCP'];
      |     SubSysCommunicationService      = [gcb,'/Communication_Service'];
      | 
      |     if strcmp(CommunicationMethod.Value, 'Ethernet TCP')
      |         set_param(SwCommunicationMethod, 'Value','0');
      | 
      |         % Set Ethernet TCP Visibilities
      |         Sw_Mode.Visible                 = 'on';
      |         EthernetTCPDescription.Visible  = 'on';
      |         set_param(SubSysEthernetTCP,'commented','off')
      | 
      |         % Set Communication Service Visibilities
      |         AdvancedSettingsContainer.Visible   = 'off';
      |         ModelStepSize.Visible               = 'off';
      |         NumSamples.Visible                  = 'off';
      |         MaxMessageSize.Visible              = 'off';
      |         COMServiceDescription.Visible       = 'off';
      |         set_param(SubSysCommunicationService,'commented','on')
      |     elseif strcmp(CommunicationMethod.Value, 'Communication Service')
      |         set_param(SwCommunicationMethod, 'Value','1');
      | 
      |         % Set Ethernet TCP Visibilities
      |         Sw_Mode.Visible                 = 'off';
      |         EthernetTCPDescription.Visible  = 'off';
      |         set_param(SubSysEthernetTCP,'commented','on')
      | 
      |         % Set Communication Service Visibilities
      |         AdvancedSettingsContainer.Visible   = 'on';
      |         ModelStepSize.Visible               = 'on';
      |         NumSamples.Visible                  = 'on';
      |         MaxMessageSize.Visible              = 'on';
      |         COMServiceDescription.Visible       = 'on';
      |         set_param(SubSysCommunicationService,'commented','off')
      |     end
      mask Callback Sw_Mode:
      | simMode     = get_param(gcb, 'Sw_Mode');
      |     subsysSIL   = [gcb,'/Ethernet_TCP/SIL'];
      |     subsysHIL   = [gcb,'/Ethernet_TCP/HIL'];
      | 
      |     if strcmp(simMode,'0') % SIL
      |         if strcmp(get_param(subsysSIL,'commented'),'on')
      |             set_param(subsysSIL,'commented','off')
      |         end
      |         if strcmp(get_param(subsysHIL,'commented'),'off')
      |             set_param(subsysHIL,'commented','on')
      |         end
      |     elseif strcmp(simMode,'1') % HIL
      |         if strcmp(get_param(subsysHIL,'commented'),'on')
      |             set_param(subsysHIL,'commented','off')
      |         end
      |         if strcmp(get_param(subsysSIL,'commented'),'off')
      |             set_param(subsysSIL,'commented','on')
      |         end
      |     else
      |         disp(['Invalid parameter value of ''', gcb, '''. Allowed values are 0 and 1'])
      |     end
      mask TypeOptions ModelStepSize: Communication_Service/dsmsi_communication_service_BL1/ModelStepSize
      mask TypeOptions NumSamples: Communication_Service/dsmsi_communication_service_BL1/NumSamples
      mask TypeOptions MaxMessageSize: Communication_Service/dsmsi_communication_service_BL1/MaxMessageSize
      mask DialogControl EthernetTCPDescription Prompt: The Ethernet TCP connection supports the following Platforms: <br> Simulation Mode <b>SIL</b>: Simulink, VEOS <br> Simulation Mode <b>HIL</b>: SCALEXIO
      mask DialogControl COMServiceDescription Prompt: For supported platforms, please refer to the help of the "ASM_COMMUNICATION_SERVICE" block.
      mask DialogControl Settings Prompt: Settings
      mask DialogControl AdvancedSettings Prompt: Advanced settings
      mask Display: disp('Configure\n Connection Settings')
  Data_Streams_Instruments : Subsystem  Tag=Animation_Data_Streams_Instruments  Priority=10001
  Fellows : Subsystem  Tag=Animation_Fellows  Priority=10001
  Lane_Sensor : Subsystem  Tag=Animation_Lane_Sensor  Priority=10001
  Lane_Sensor_Dynamic_Instruments : Subsystem  Tag=Animation_Lane_Sensor_Dynamic_Instruments  Priority=10001  Commented=on
  Sensors : Subsystem  Tag=Animation_Sensors  Priority=10001
  Sw_Sensor_Animation[] : Constant
      settings: AttributesFormatString=1_Object3D\n2_Object2D\n3_TrafficSign\n4_LineSensor_Road_Lanes\n5_LineSensor_Road_Shape_Lines\n6_LineSensor_Road_Shape_ContObj\n7_LineSensor_Junction_Borders\n8_LineSensor_Junction_Shape_Lines\n9_LineSensor_Junction_Shape_ContObj\n10_Object3D_RadarEffects\n11_Object3D_CustomPoints
  Sw_Sensor_Selector[] : Constant
  wires:
  Environment_Animation/1 -> ASM_Vehicle_Instruments/2(Environment_Animation), Connection_Settings/1(Environment_Animation), Lane_Sensor_Dynamic_Instruments/1(Environment_Animation), Lane_Sensor/1(Environment_Animation), Fellows/1(Environment_Animation), Data_Streams_Instruments/1(Environment_Animation), Bounding_Boxes/1(Environment_Animation), Sensors/4(Environment_Animation), ASM_Vehicle_Occupants/1(Environment_Animation)
  Fellow_Doors/1 -> Fellows/3(Fellow_Doors)
  ASM_Vehicle_Doors/1 -> ASM_Vehicle/3(ASM_Vehicle_Doors)
  ASM_Vehicle_Lights/1 -> ASM_Vehicle/1(ASM_Vehicle_Lights)
  Fellow_Lights/1 -> Fellows/2(Fellow_Lights)
  Sw_Sensor_Selector[]/1 -> Sensors/2(Sw_Sensor_Selector[])
  Sw_Sensor_Animation[]/1 -> Sensors/3(Sw_Sensor_Animation[])
  Drivetrain_Animation/1 -> ASM_Vehicle_Instruments/3(Drivetrain_Animation)
  ASM_Vehicle/1(Chassis_Transformation_Matrix) -> Sensors/1(Transform_In)
  VehicleDynamics_Animation/1 -> ASM_Vehicle/2(VehicleDynamics_Animation), ASM_Vehicle_Instruments/1(VehicleDynamics_Animation)
  DriverAssistance_Animation/1 -> ACC_Instruments/1(DriverAssistance_Animation)

== system ASM_Traffic_MultiCore/AnimationInterface/FcnCall ==
  ManeuverState[] : Inport
  Enable1 : EnablePort
  Disable : Constant  Value=0  OutDataTypeStr=Inherit: Inherit via back propagation
  Enable : Constant  OutDataTypeStr=Inherit: Inherit via back propagation
  External_Samples : Subsystem  TreatAsAtomicUnit=on  SystemSampleTime=SIM.StepSize.v
      settings: AttributesFormatString=Ts=%<SystemSampleTime>
  MANEUVER_FCN_CALL_GENERATOR : ASM_Environment_lib/Environment/Maneuver/MANEUVER_FCN_CALL_GENERATOR  NumSamples=SIM.NumSamplesAnimation.v  ASMProperties=struct('Name','MANEUVER_FCN_CALL_GENERATOR','Version','3.0','Library','ASM_Environment_lib')  ASMInstanceName=maneuver_fcn_call_generator  ASMInstanceID=1
  Samples_Ext[] : Constant  OutDataTypeStr=Inherit: Inherit via back propagation
  Switch : Switch  Criteria=u2 ~= 0  SaturateOnIntegerOverflow=off  InputSameDT=off
  Switch1 : Switch  Criteria=u2 ~= 0  SaturateOnIntegerOverflow=off  InputSameDT=off
  Valid_Samples : simulink/Logic and Bit Operations/Compare To Zero  relop=>  OutDataTypeStr=boolean
  FcnCallEvent[] : Outport
  wires:
  External_Samples/1(num_Samples[]) -> Valid_Samples/1, Switch/1
  Valid_Samples/1 -> Switch1/2, Switch/2
  Switch/1 -> MANEUVER_FCN_CALL_GENERATOR/3
  Switch1/1 -> MANEUVER_FCN_CALL_GENERATOR/2
  Samples_Ext[]/1 -> Switch/3
  Enable/1 -> Switch1/1
  ManeuverState[]/1 -> MANEUVER_FCN_CALL_GENERATOR/1
  MANEUVER_FCN_CALL_GENERATOR/1 -> FcnCallEvent[]/1
  Disable/1 -> Switch1/3
